simulink model "QD2_Sim_Dual"  (R2025a)
settings: Solver=FixedStepDiscrete  StartTime=0.0  StopTime=400  FixedStep=0.002  RelTol=1e-3
PreLoadFcn:
  | % QD2_Sim_Dual: agrega lib/ y sim/ al path antes de cargar (enlaces a QD2_Mission_Lib)
  | qd2_c = {pwd};
  | qd2_w = which('QD2_Sim_Dual');
  | if ~isempty(qd2_w), qd2_c{end+1} = fileparts(qd2_w); end
  | for qd2_i = 1:numel(qd2_c)
  |     qd2_d = qd2_c{qd2_i};
  |     for qd2_k = 1:4
  |         if exist(fullfile(qd2_d, 'lib', 'QD2_Mission_Lib.slx'), 'file')
  |             addpath(fullfile(qd2_d, 'lib'));
  |             addpath(fullfile(qd2_d, 'sim'));
  |             break;
  |         end
  |         qd2_d = fileparts(qd2_d);
  |     end
  | end
  | clear qd2_c qd2_w qd2_i qd2_d qd2_k
PostLoadFcn:
  | % QD2_Sim_Dual: rutas de lib/ (funciones qd2_* y QD2_Mission_Lib) y sim/
  | qd2_d = fileparts(get_param(bdroot, 'FileName'));
  | for qd2_k = 1:4
  |     if exist(fullfile(qd2_d, 'lib', 'qd2_params.m'), 'file'), break; end
  |     qd2_d = fileparts(qd2_d);
  | end
  | addpath(fullfile(qd2_d, 'lib'));
  | addpath(fullfile(qd2_d, 'sim'));
  | clear qd2_d qd2_k
InitFcn:
  | % QD2_Sim_Dual: rutas de lib/ (funciones qd2_* y QD2_Mission_Lib) y sim/
  | qd2_d = fileparts(get_param(bdroot, 'FileName'));
  | for qd2_k = 1:4
  |     if exist(fullfile(qd2_d, 'lib', 'qd2_params.m'), 'file'), break; end
  |     qd2_d = fileparts(qd2_d);
  | end
  | addpath(fullfile(qd2_d, 'lib'));
  | addpath(fullfile(qd2_d, 'sim'));
  | clear qd2_d qd2_k
  | % Parámetros (config/estacion.json es la única fuente de verdad)
  | QD2P = qd2_params_from_config();
  | QD2_SIM = qd2_sim_parametros();
  | % La versión la fija el bloque constante VERSION de la raíz
  | QD2_VERSION = str2double(get_param([bdroot '/' sprintf('VERSION\n(1 = PID, 2 = MPC)')], 'Value'));
libraries: QD2_Mission_Lib x11, quarc_library x2, simulink x1
settings Model: ExtModeTrigDuration=10000  Creator=ezequ  LastModifiedBy=ezequ
settings SolverCC: AlgebraicLoopSolver=TrustRegion  PositivePriorityOrder=on
settings DataIOCC: SaveFormat=Array  SaveOutput=off  SignalLogging=off  SaveTime=off
settings OptimizationCC: LifeSpan=inf
settings DebuggingCC: AlgebraicLoopMsg=error  UnconnectedInputMsg=warning  UnconnectedOutputMsg=warning  UnconnectedLineMsg=warning  ArithmeticOperatorsInVariantConditions=warning
settings ModelReferenceCC: EnableRefExpFcnMdlSchedulingChecks=on
settings SFSimCC: SimUseLocalCustomCode=off  CustomCodeUndefinedFunction=UseInterfaceOnly
settings RTWCC: SystemTargetFile=quarc_win64.tlc  TemplateMakefile=quarc_default_tmf  RTWUseLocalCustomCode=off  GPUComputeCapability=3.5  Description=QUARC Win64 Target
settings CodeAppCC: StateflowObjectComments=on
settings STFCustomTargetCC: SystemTargetFile=quarc_win64.tlc  TargetPreCompLibLocation=C:\PROGRA~3\QUARC\lib\2016a\win64\release  TargetLangStandard=C99 (ISO)  MultiwordLength=2048.0  DynamicStringBufferSize=256.0  ConcurrentExecutionCompliant=on  Debug=off  StopOnOverrun=off  DownloadToTarget=on
settings GRTTargetCC: ExtMode=on  ExtModeMexFile=quarc_comm  TargetPreCompLibLocation=C:\PROGRA~3\QUARC\lib\2016a\win64\release  ParMdlRefBuildCompliant=off  CompOptLevelCompliant=off  CombineOutputUpdateFcns=off  MatFileLogging=off  CPPClassGenCompliant=off  GRTInterface=on  UseToolchainInfoCompliant=off
settings ConfigComp: CovMetricSettings=dswe

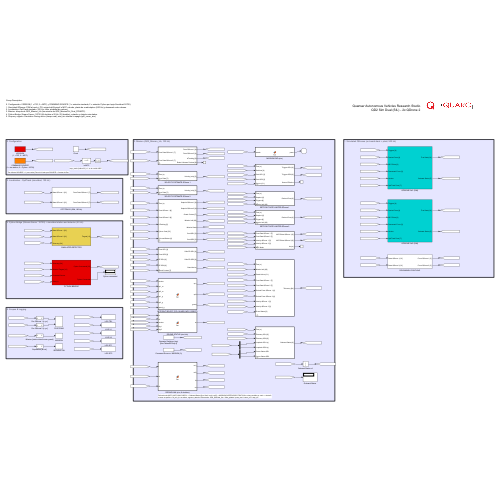
[thumbnail: Simulink's stored preview of the top-level diagram]
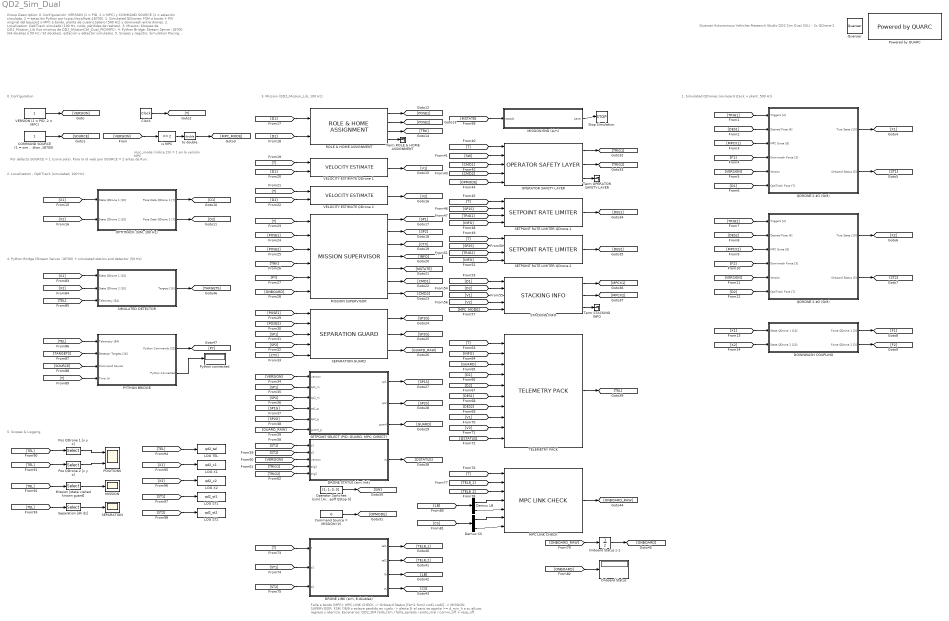
== system QD2_Sim_Dual ==
  note: Group Description:
      |
      | 0. Configuración: VERSION (1 = PID, 2 = MPC) y COMMAND SOURCE (1 = estación simulada, 2 = estación Python por tcpip://localhost:18700).
      | 1. Simulated QDrones: FSM a bordo + PIV original del Equipo2 o MPC a bordo, planta de cuadricóptero (500 Hz) y downwash entre drones.
      | 2. Localization: OptiTrack simulado (100 Hz, ruido, pérdidas de rastreo).
      | 3. Mission: bloques de QD2_Mission_Lib (los mismos de QD2_MissionCtrl_Dual_PID/MPC).
      | 4. Python Bridge: Stream Server :18700 (64 doubles a 50 Hz / 32 doubles), estación y detector simulados.
      | 5. Scopes y registro. Simulation Pacing activo (tiempo real); sim() sin interfaz lo apaga (qd2_correr_sim).
  note: Quanser Autonomous Vehicles Research Studio
      | QD2 Sim Dual (SIL) - 2x QDrone 2
  note: 0. Configuration
  note: mpc_mode (índice 23) = 1 en la versión MPC
  note: Por defecto SOURCE = 1 (corre sola). Para la UI web pon SOURCE = 2 antes de Run.
  note: 1. Simulated QDrones (on-board stack + plant, 500 Hz)
  note: 2. Localization - OptiTrack (simulated, 100 Hz)
  note: 3. Mission (QD2_Mission_Lib, 100 Hz)
  note: Falla a bordo (MPC): MPC LINK CHECK -> Onboard Status [fsm1 fsm2 cod1 cod2] -> MISSION SUPERVISOR. FSM 7/8/9 o enlace perdido en vuelo -> alerta 9:
      | el sano se aparta >= d_min_h a su altura, regresa y aterriza. Escenarios: QD2_SIM.falla_fsm / falla_apilado / proto_mal / comm_off + resp_off.
  note: 4. Python Bridge (Stream Server :18700) + simulated station and detector (50 Hz)
  note: 5. Scopes & Logging
  "COMMAND SOURCE (1 = sim station, 2 = Python :18700)" : Constant
  Clock : DigitalClock  SampleTime=0.01
  Command Source = MISSION (0) : Constant  Value=0  SampleTime=0.01
  DOWNWASH COUPLING : Subsystem
  "DRONE LINK (sim, 8 doubles)" : MATLAB Function  TreatAsAtomicUnit=on
  DRONE STATUS (sim link) : MATLAB Function  TreatAsAtomicUnit=on
  Demux CS : Demux  Outputs=2
  Demux LB : Demux  Outputs=2
  LOG ST1 : ToWorkspace  VariableName=qd2_st1  SampleTime=0.02
  LOG ST2 : ToWorkspace  VariableName=qd2_st2  SampleTime=0.02
  LOG TEL : ToWorkspace  VariableName=qd2_tel  SampleTime=0.02
  LOG X1 : ToWorkspace  VariableName=qd2_x1  SampleTime=0.02
  LOG X2 : ToWorkspace  VariableName=qd2_x2  SampleTime=0.02
  MISSION : Scope
  MISSION END (sim) : MATLAB Function  TreatAsAtomicUnit=on
  MISSION SUPERVISOR : QD2_Mission_Lib/MISSION SUPERVISOR  P=QD2P  version=QD2_VERSION  Ts=0.01
  MPC LINK CHECK : QD2_Mission_Lib/MPC LINK CHECK  P=QD2P  version=QD2_VERSION  Ts=0.01
  Mission [state visited known guard] : Selector  InputPortWidth=64  IndexOptions=Index vector (dialog)  Indices=[2 10 9 11]  OutputSizes=1
  OPERATOR SAFETY LAYER : QD2_Mission_Lib/OPERATOR SAFETY LAYER  Ts=0.01
  "OPTITRACK (SIM, 100 Hz)" : Subsystem
  Onboard Status : Display
  Onboard Status z-1 : UnitDelay  InitialCondition=[0; 0; 0; 0]  SampleTime=0.01  HasFrameUpgradeWarning=on
  Operator Switches (sim) [Arm Takeoff EStop 0] : Constant  Value=[1; 1; 0; 0]  SampleTime=0.01
  POSITIONS : Scope  NumInputPorts=2
  PYTHON BRIDGE : Subsystem
  Pos QDrone 1 [x y z] : Selector  InputPortWidth=64  IndexOptions=Index vector (dialog)  Indices=[17 18 19]  OutputSizes=1
  Pos QDrone 2 [x y z] : Selector  InputPortWidth=64  IndexOptions=Index vector (dialog)  Indices=[35 36 37]  OutputSizes=1
  Powered by QUARC : quarc_library/Logos/Powered by QUARC
  Python connected : Display
  QDRONE 2 #1 (SIM) : Subsystem
  QDRONE 2 #2 (SIM) : Subsystem
  Quanser : quarc_library/Logos/Quanser
  ROLE & HOME ASSIGNMENT : QD2_Mission_Lib/ROLE & HOME ASSIGNMENT  P=QD2P  version=QD2_VERSION  Ts=0.01
  SEPARATION : Scope
  SEPARATION GUARD : QD2_Mission_Lib/SEPARATION GUARD  P=QD2P  Ts=0.01
  SETPOINT RATE LIMITER QDrone 1 : QD2_Mission_Lib/SETPOINT RATE LIMITER  P=QD2P  dron=1  Ts=0.01
  SETPOINT RATE LIMITER QDrone 2 : QD2_Mission_Lib/SETPOINT RATE LIMITER  P=QD2P  dron=2  Ts=0.01
  "SETPOINT SELECT (PID: GUARD, MPC: DIRECT)" : MATLAB Function  TreatAsAtomicUnit=on
  SIMULATED DETECTOR : Subsystem
  STACKING INFO : QD2_Mission_Lib/STACKING INFO  Ts=0.01
  Separation [dh dz] : Selector  InputPortWidth=64  IndexOptions=Index vector (dialog)  Indices=[12 13]  OutputSizes=1
  Stop Simulation : Stop
  TELEMETRY PACK : QD2_Mission_Lib/TELEMETRY PACK  version=QD2_VERSION  Ts=0.01
  Term OPERATOR SAFETY LAYER : Terminator
  Term ROLE & HOME ASSIGNMENT : Terminator
  Term STACKING INFO : Terminator
  VELOCITY ESTIMATE QDrone 1 : QD2_Mission_Lib/VELOCITY ESTIMATE  Ts=0.01
  VELOCITY ESTIMATE QDrone 2 : QD2_Mission_Lib/VELOCITY ESTIMATE  Ts=0.01
  "VERSION (1 = PID, 2 = MPC)" : Constant
  is MPC : simulink/Logic and Bit Operations/Compare To Constant  relop===  const=2  OutDataTypeStr=boolean
  to double : DataTypeConversion  OutDataTypeStr=double  SaturateOnIntegerOverflow=off  RndMeth=Floor
  wires:
  "VERSION (1 = PID, 2 = MPC)"/1 -> [VERSION]
  "COMMAND SOURCE (1 = sim station, 2 = Python :18700)"/1 -> [SOURCE]
  Clock/1 -> [T]
  is MPC/1 -> to double/1
  [VERSION] -> is MPC/1
  to double/1 -> [MPC_MODE]
  [TRIG1] -> QDRONE 2 #1 (SIM)/1(Triggers [4])
  [DES1] -> QDRONE 2 #1 (SIM)/2(Desired Pose [4])
  [MPCX1] -> QDRONE 2 #1 (SIM)/3(MPC Extra [8])
  [F1] -> QDRONE 2 #1 (SIM)/4(Downwash Force [3])
  [VERSION] -> QDRONE 2 #1 (SIM)/5(Version)
  [D1] -> QDRONE 2 #1 (SIM)/6(OptiTrack Pose [7])
  QDRONE 2 #1 (SIM)/1(True State [10]) -> [X1]
  QDRONE 2 #1 (SIM)/2(Onboard Status [5]) -> [ST1]
  [TRIG2] -> QDRONE 2 #2 (SIM)/1(Triggers [4])
  [DES2] -> QDRONE 2 #2 (SIM)/2(Desired Pose [4])
  [MPCX2] -> QDRONE 2 #2 (SIM)/3(MPC Extra [8])
  [F2] -> QDRONE 2 #2 (SIM)/4(Downwash Force [3])
  [VERSION] -> QDRONE 2 #2 (SIM)/5(Version)
  [D2] -> QDRONE 2 #2 (SIM)/6(OptiTrack Pose [7])
  QDRONE 2 #2 (SIM)/1(True State [10]) -> [X2]
  QDRONE 2 #2 (SIM)/2(Onboard Status [5]) -> [ST2]
  [X1] -> DOWNWASH COUPLING/1(State QDrone 1 [10])
  [X2] -> DOWNWASH COUPLING/2(State QDrone 2 [10])
  DOWNWASH COUPLING/1(Force QDrone 1 [3]) -> [F1]
  DOWNWASH COUPLING/2(Force QDrone 2 [3]) -> [F2]
  [X1] -> "OPTITRACK (SIM, 100 Hz)"/1(State QDrone 1 [10])
  [X2] -> "OPTITRACK (SIM, 100 Hz)"/2(State QDrone 2 [10])
  "OPTITRACK (SIM, 100 Hz)"/1(Pose Data QDrone 1 [7]) -> [D1]
  "OPTITRACK (SIM, 100 Hz)"/2(Pose Data QDrone 2 [7]) -> [D2]
  [D1] -> ROLE & HOME ASSIGNMENT/1
  [D2] -> ROLE & HOME ASSIGNMENT/2
  ROLE & HOME ASSIGNMENT/1 -> [POSE1]
  ROLE & HOME ASSIGNMENT/2 -> [POSE2]
  ROLE & HOME ASSIGNMENT/3 -> [TRK]
  ROLE & HOME ASSIGNMENT/4 -> Term ROLE & HOME ASSIGNMENT/1
  [T] -> VELOCITY ESTIMATE QDrone 1/1
  [D1] -> VELOCITY ESTIMATE QDrone 1/2
  VELOCITY ESTIMATE QDrone 1/1 -> [V1]
  [T] -> VELOCITY ESTIMATE QDrone 2/1
  [D2] -> VELOCITY ESTIMATE QDrone 2/2
  VELOCITY ESTIMATE QDrone 2/1 -> [V2]
  [T] -> MISSION SUPERVISOR/1
  [POSE1] -> MISSION SUPERVISOR/2
  [POSE2] -> MISSION SUPERVISOR/3
  [TRK] -> MISSION SUPERVISOR/4
  [PY] -> MISSION SUPERVISOR/5
  [ONBOARD] -> MISSION SUPERVISOR/6
  MISSION SUPERVISOR/1 -> [SP1]
  MISSION SUPERVISOR/2 -> [SP2]
  MISSION SUPERVISOR/3 -> [CTX]
  MISSION SUPERVISOR/4 -> [INFO]
  MISSION SUPERVISOR/5 -> [MSTATE]
  MISSION SUPERVISOR/6 -> [CMD1]
  MISSION SUPERVISOR/7 -> [CMD2]
  [POSE1] -> SEPARATION GUARD/1
  [POSE2] -> SEPARATION GUARD/2
  [SP1] -> SEPARATION GUARD/3
  [SP2] -> SEPARATION GUARD/4
  [CTX] -> SEPARATION GUARD/5
  SEPARATION GUARD/1 -> [SP1G]
  SEPARATION GUARD/2 -> [SP2G]
  SEPARATION GUARD/3 -> [GUARD_RAW]
  [VERSION] -> "SETPOINT SELECT (PID: GUARD, MPC: DIRECT)"/1(version)
  [SP1] -> "SETPOINT SELECT (PID: GUARD, MPC: DIRECT)"/2(sp1_m)
  [SP2] -> "SETPOINT SELECT (PID: GUARD, MPC: DIRECT)"/3(sp2_m)
  [SP1G] -> "SETPOINT SELECT (PID: GUARD, MPC: DIRECT)"/4(sp1_g)
  [SP2G] -> "SETPOINT SELECT (PID: GUARD, MPC: DIRECT)"/5(sp2_g)
  [GUARD_RAW] -> "SETPOINT SELECT (PID: GUARD, MPC: DIRECT)"/6(guard_g)
  "SETPOINT SELECT (PID: GUARD, MPC: DIRECT)"/1(sp1) -> [SP1S]
  "SETPOINT SELECT (PID: GUARD, MPC: DIRECT)"/2(sp2) -> [SP2S]
  "SETPOINT SELECT (PID: GUARD, MPC: DIRECT)"/3(guard) -> [GUARD]
  Operator Switches (sim) [Arm Takeoff EStop 0]/1 -> [SW]
  Command Source = MISSION (0)/1 -> [OPMODE]
  [T] -> OPERATOR SAFETY LAYER/1
  [SW] -> OPERATOR SAFETY LAYER/2
  [CMD1] -> OPERATOR SAFETY LAYER/3
  [CMD2] -> OPERATOR SAFETY LAYER/4
  [OPMODE] -> OPERATOR SAFETY LAYER/5
  OPERATOR SAFETY LAYER/1 -> [TRIG1]
  OPERATOR SAFETY LAYER/2 -> [TRIG2]
  OPERATOR SAFETY LAYER/3 -> Term OPERATOR SAFETY LAYER/1
  [T] -> SETPOINT RATE LIMITER QDrone 1/1
  [SP1S] -> SETPOINT RATE LIMITER QDrone 1/2
  [TRIG1] -> SETPOINT RATE LIMITER QDrone 1/3
  [INFO] -> SETPOINT RATE LIMITER QDrone 1/4
  SETPOINT RATE LIMITER QDrone 1/1 -> [DES1]
  [T] -> SETPOINT RATE LIMITER QDrone 2/1
  [SP2S] -> SETPOINT RATE LIMITER QDrone 2/2
  [TRIG2] -> SETPOINT RATE LIMITER QDrone 2/3
  [INFO] -> SETPOINT RATE LIMITER QDrone 2/4
  SETPOINT RATE LIMITER QDrone 2/1 -> [DES2]
  [D1] -> STACKING INFO/1
  [D2] -> STACKING INFO/2
  [V1] -> STACKING INFO/3
  [V2] -> STACKING INFO/4
  [MPC_MODE] -> STACKING INFO/5
  STACKING INFO/1 -> [MPCX1]
  STACKING INFO/2 -> [MPCX2]
  STACKING INFO/3 -> Term STACKING INFO/1
  [ST1] -> DRONE STATUS (sim link)/1(s1)
  [ST2] -> DRONE STATUS (sim link)/2(s2)
  [VERSION] -> DRONE STATUS (sim link)/3(version)
  [TRIG1] -> DRONE STATUS (sim link)/4(trig1)
  [TRIG2] -> DRONE STATUS (sim link)/5(trig2)
  DRONE STATUS (sim link)/1(st) -> [DSTATUS]
  [T] -> TELEMETRY PACK/1
  [INFO] -> TELEMETRY PACK/2
  [GUARD] -> TELEMETRY PACK/3
  [D1] -> TELEMETRY PACK/4
  [D2] -> TELEMETRY PACK/5
  [DES1] -> TELEMETRY PACK/6
  [DES2] -> TELEMETRY PACK/7
  [V1] -> TELEMETRY PACK/8
  [V2] -> TELEMETRY PACK/9
  [DSTATUS] -> TELEMETRY PACK/10
  TELEMETRY PACK/1 -> [TEL]
  [T] -> "DRONE LINK (sim, 8 doubles)"/1(t)
  [ST1] -> "DRONE LINK (sim, 8 doubles)"/2(s1)
  [ST2] -> "DRONE LINK (sim, 8 doubles)"/3(s2)
  "DRONE LINK (sim, 8 doubles)"/1(tel1) -> [TEL8_1]
  "DRONE LINK (sim, 8 doubles)"/2(tel2) -> [TEL8_2]
  "DRONE LINK (sim, 8 doubles)"/3(lb) -> [LB]
  "DRONE LINK (sim, 8 doubles)"/4(cs) -> [CS]
  [T] -> MPC LINK CHECK/1
  [TEL8_1] -> MPC LINK CHECK/2
  [TEL8_2] -> MPC LINK CHECK/3
  MPC LINK CHECK/1 -> [ONBOARD_RAW]
  [ONBOARD_RAW] -> Onboard Status z-1/1
  Onboard Status z-1/1 -> [ONBOARD]
  [LB] -> Demux LB/1
  Demux LB/1 -> MPC LINK CHECK/4
  Demux LB/2 -> MPC LINK CHECK/5
  [CS] -> Demux CS/1
  Demux CS/1 -> MPC LINK CHECK/6
  Demux CS/2 -> MPC LINK CHECK/7
  [ONBOARD] -> Onboard Status/1
  [X1] -> SIMULATED DETECTOR/1(State QDrone 1 [10])
  [X2] -> SIMULATED DETECTOR/2(State QDrone 2 [10])
  [TEL] -> SIMULATED DETECTOR/3(Telemetry [64])
  SIMULATED DETECTOR/1(Targets [16]) -> [TARGETS]
  [TEL] -> PYTHON BRIDGE/1(Telemetry [64])
  [TARGETS] -> PYTHON BRIDGE/2(Detector Targets [16])
  [SOURCE] -> PYTHON BRIDGE/3(Command Source)
  [T] -> PYTHON BRIDGE/4(Time (s))
  PYTHON BRIDGE/1(Python Commands [32]) -> [PY]
  PYTHON BRIDGE/2(Python Connected) -> Python connected/1
  [TEL] -> Pos QDrone 1 [x y z]/1
  [TEL] -> Pos QDrone 2 [x y z]/1
  [TEL] -> Mission [state visited known guard]/1
  [TEL] -> Separation [dh dz]/1
  Pos QDrone 1 [x y z]/1 -> POSITIONS/1
  Pos QDrone 2 [x y z]/1 -> POSITIONS/2
  Mission [state visited known guard]/1 -> MISSION/1
  Separation [dh dz]/1 -> SEPARATION/1
  [TEL] -> LOG TEL/1
  [X1] -> LOG X1/1
  [X2] -> LOG X2/1
  [ST1] -> LOG ST1/1
  [ST2] -> LOG ST2/1
  [MSTATE] -> MISSION END (sim)/1(estado)
  MISSION END (sim)/1(parar) -> Stop Simulation/1

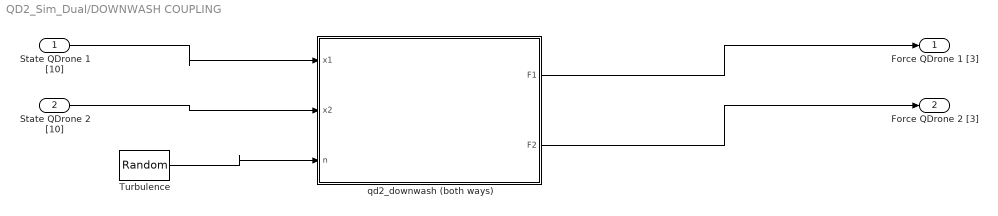
== system QD2_Sim_Dual/DOWNWASH COUPLING ==
  State QDrone 1 [10] : Inport
  State QDrone 2 [10] : Inport  Port=2
  Turbulence : RandomNumber  Mean=zeros(6,1)  Variance=ones(6,1)  Seed=QD2_SIM.semilla + [11 12 13 14 15 16]'  SampleTime=0.002
  qd2_downwash (both ways) : MATLAB Function  TreatAsAtomicUnit=on
  Force QDrone 1 [3] : Outport
  Force QDrone 2 [3] : Outport  Port=2
  wires:
  State QDrone 1 [10]/1 -> qd2_downwash (both ways)/1(x1)
  State QDrone 2 [10]/1 -> qd2_downwash (both ways)/2(x2)
  Turbulence/1 -> qd2_downwash (both ways)/3(n)
  qd2_downwash (both ways)/1(F1) -> Force QDrone 1 [3]/1
  qd2_downwash (both ways)/2(F2) -> Force QDrone 2 [3]/1

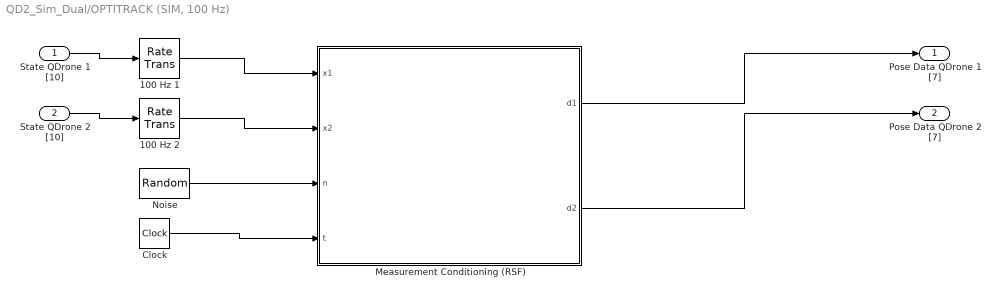
== system QD2_Sim_Dual/OPTITRACK (SIM, 100 Hz) ==
  State QDrone 1 [10] : Inport
  State QDrone 2 [10] : Inport  Port=2
  100 Hz 1 : RateTransition  OutPortSampleTime=0.01
  100 Hz 2 : RateTransition  OutPortSampleTime=0.01
  Clock : DigitalClock  SampleTime=0.01
  Measurement Conditioning (RSF) : MATLAB Function  TreatAsAtomicUnit=on
  Noise : RandomNumber  Mean=zeros(8,1)  Variance=ones(8,1)  Seed=QD2_SIM.semilla + (21:28)'  SampleTime=0.01
  Pose Data QDrone 1 [7] : Outport
  Pose Data QDrone 2 [7] : Outport  Port=2
  wires:
  State QDrone 1 [10]/1 -> 100 Hz 1/1
  State QDrone 2 [10]/1 -> 100 Hz 2/1
  100 Hz 1/1 -> Measurement Conditioning (RSF)/1(x1)
  100 Hz 2/1 -> Measurement Conditioning (RSF)/2(x2)
  Noise/1 -> Measurement Conditioning (RSF)/3(n)
  Clock/1 -> Measurement Conditioning (RSF)/4(t)
  Measurement Conditioning (RSF)/1(d1) -> Pose Data QDrone 1 [7]/1
  Measurement Conditioning (RSF)/2(d2) -> Pose Data QDrone 2 [7]/1

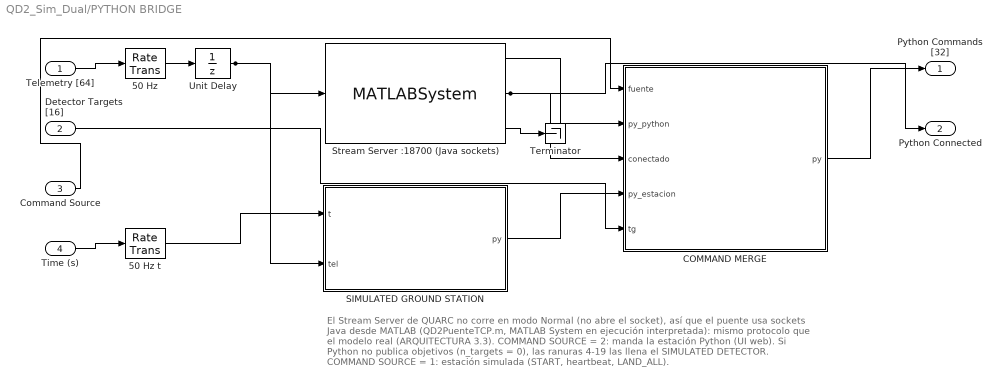
== system QD2_Sim_Dual/PYTHON BRIDGE ==
  note: El Stream Server de QUARC no corre en modo Normal (no abre el socket), así que el puente usa sockets Java desde MATLAB
      | (QD2PuenteTCP.m, MATLAB System en ejecución interpretada): mismo protocolo que el modelo real (ARQUITECTURA 3.3).
      | COMMAND SOURCE = 2: manda la estación Python (UI web). Si Python no publica objetivos (n_targets = 0), las
      | ranuras 4-19 las llena el SIMULATED DETECTOR. COMMAND SOURCE = 1: estación simulada (START, heartbeat, LAND_ALL).
  Telemetry [64] : Inport
  Detector Targets [16] : Inport  Port=2
  Command Source : Inport  Port=3
  Time (s) : Inport  Port=4
  50 Hz : RateTransition  OutPortSampleTime=0.02
  50 Hz t : RateTransition  OutPortSampleTime=0.02
  COMMAND MERGE : MATLAB Function  TreatAsAtomicUnit=on
  SIMULATED GROUND STATION : MATLAB Function  TreatAsAtomicUnit=on
  Stream Server :18700 (Java sockets) : MATLABSystem  System=QD2PuenteTCP  Puerto=QD2_SIM.puerto  Direccion=127.0.0.1  Activo=1  TDesconectar=5  Ts=0.02
      mask Type: QD2PuenteTCP
  Terminator : Terminator
  Unit Delay : UnitDelay  InitialCondition=zeros(64,1)  SampleTime=0.02  HasFrameUpgradeWarning=on
  Python Commands [32] : Outport
  Python Connected : Outport  Port=2
  wires:
  Telemetry [64]/1 -> 50 Hz/1
  50 Hz/1 -> Unit Delay/1
  Unit Delay/1 -> Stream Server :18700 (Java sockets)/1, SIMULATED GROUND STATION/2(tel)
  Time (s)/1 -> 50 Hz t/1
  50 Hz t/1 -> SIMULATED GROUND STATION/1(t)
  Command Source/1 -> COMMAND MERGE/1(fuente)
  Stream Server :18700 (Java sockets)/1 -> COMMAND MERGE/2(py_python)
  Stream Server :18700 (Java sockets)/2 -> COMMAND MERGE/3(conectado), Python Connected/1
  SIMULATED GROUND STATION/1(py) -> COMMAND MERGE/4(py_estacion)
  Detector Targets [16]/1 -> COMMAND MERGE/5(tg)
  COMMAND MERGE/1(py) -> Python Commands [32]/1
  Stream Server :18700 (Java sockets)/3 -> Terminator/1

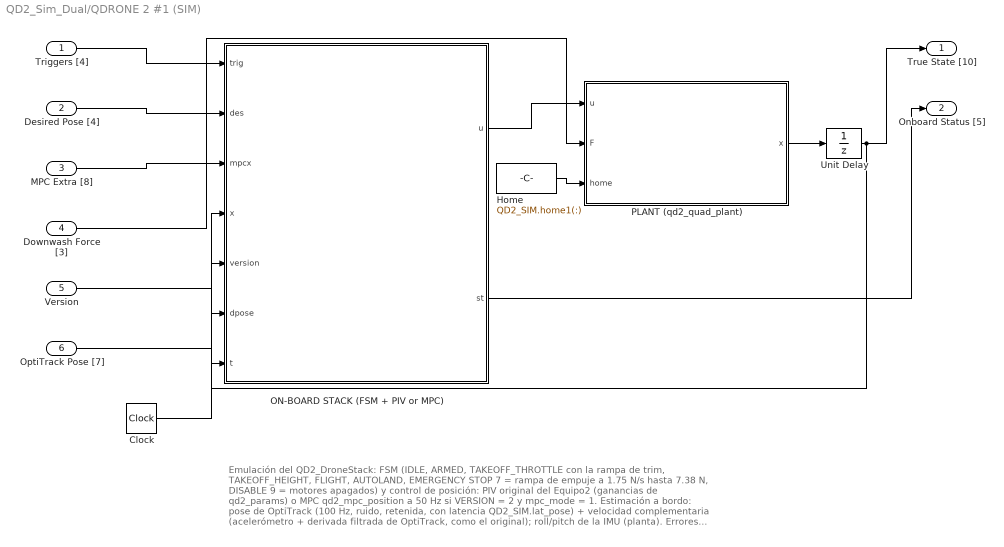
== system QD2_Sim_Dual/QDRONE 2 #1 (SIM) ==
  note: Emulación del QD2_DroneStack: FSM (IDLE, ARMED, TAKEOFF_THROTTLE con la rampa de trim, TAKEOFF_HEIGHT, FLIGHT, AUTOLAND,
      | EMERGENCY STOP 7 = rampa de empuje a 1.75 N/s hasta 7.38 N, DISABLE 9 = motores apagados) y control de posición: PIV original del
      | Equipo2 (ganancias de qd2_params) o MPC qd2_mpc_position a 50 Hz si VERSION = 2 y mpc_mode = 1.
      | Estimación a bordo: pose de OptiTrack (100 Hz, ruido, retenida, con latencia QD2_SIM.lat_pose) + velocidad complementaria
      | (acelerómetro + derivada filtrada de OptiTrack, como el original); roll/pitch de la IMU (planta). Errores como el original:
      | isTracking = 0 durante 0.2 s -> 7; enlace caído (QD2_SIM.comm_off) 0.5 s -> 7 y 1 s armado -> 9 (FLIGHT SAFETY corta motores).
      | Fallas a bordo programadas: QD2_SIM.falla_fsm [dron t] o QD2_SIM.falla_apilado (1 = el de arriba, 2 = el de abajo) -> 7.
      | Onboard Status = [FSM, batería (V), estado MPC (0 ok, 3 inactivo, 4 PIV), empuje (N), comm issue].
      | True State = [x y z vx vy vz roll pitch yaw T]. El STABILIZER se aproxima con la actitud de 1er orden de la planta.
  Triggers [4] : Inport
  Desired Pose [4] : Inport  Port=2
  MPC Extra [8] : Inport  Port=3
  Downwash Force [3] : Inport  Port=4
  Version : Inport  Port=5
  OptiTrack Pose [7] : Inport  Port=6
  Clock : DigitalClock  SampleTime=0.002
  Home : Constant  Value=QD2_SIM.home1(:)
  ON-BOARD STACK (FSM + PIV or MPC) : MATLAB Function  TreatAsAtomicUnit=on
  PLANT (qd2_quad_plant) : MATLAB Function  TreatAsAtomicUnit=on
  Unit Delay : UnitDelay  InitialCondition=[QD2_SIM.home1(:); zeros(8,1)]  SampleTime=0.002  HasFrameUpgradeWarning=on
  True State [10] : Outport
  Onboard Status [5] : Outport  Port=2
  wires:
  Triggers [4]/1 -> ON-BOARD STACK (FSM + PIV or MPC)/1(trig)
  Desired Pose [4]/1 -> ON-BOARD STACK (FSM + PIV or MPC)/2(des)
  MPC Extra [8]/1 -> ON-BOARD STACK (FSM + PIV or MPC)/3(mpcx)
  Unit Delay/1 -> ON-BOARD STACK (FSM + PIV or MPC)/4(x), True State [10]/1
  Version/1 -> ON-BOARD STACK (FSM + PIV or MPC)/5(version)
  OptiTrack Pose [7]/1 -> ON-BOARD STACK (FSM + PIV or MPC)/6(dpose)
  Clock/1 -> ON-BOARD STACK (FSM + PIV or MPC)/7(t)
  ON-BOARD STACK (FSM + PIV or MPC)/1(u) -> PLANT (qd2_quad_plant)/1(u)
  Downwash Force [3]/1 -> PLANT (qd2_quad_plant)/2(F)
  Home/1 -> PLANT (qd2_quad_plant)/3(home)
  PLANT (qd2_quad_plant)/1(x) -> Unit Delay/1
  ON-BOARD STACK (FSM + PIV or MPC)/2(st) -> Onboard Status [5]/1

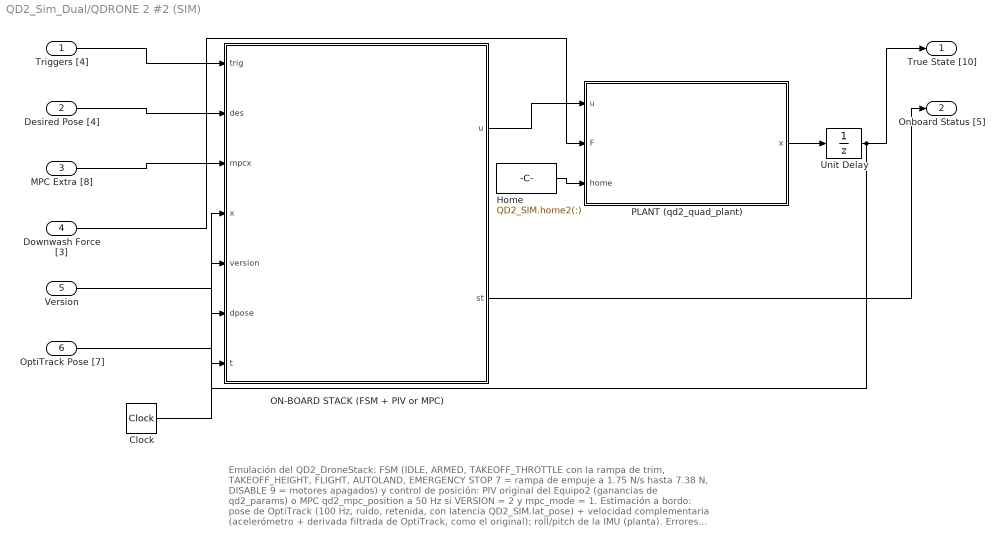
== system QD2_Sim_Dual/QDRONE 2 #2 (SIM) ==
  note: Emulación del QD2_DroneStack: FSM (IDLE, ARMED, TAKEOFF_THROTTLE con la rampa de trim, TAKEOFF_HEIGHT, FLIGHT, AUTOLAND,
      | EMERGENCY STOP 7 = rampa de empuje a 1.75 N/s hasta 7.38 N, DISABLE 9 = motores apagados) y control de posición: PIV original del
      | Equipo2 (ganancias de qd2_params) o MPC qd2_mpc_position a 50 Hz si VERSION = 2 y mpc_mode = 1.
      | Estimación a bordo: pose de OptiTrack (100 Hz, ruido, retenida, con latencia QD2_SIM.lat_pose) + velocidad complementaria
      | (acelerómetro + derivada filtrada de OptiTrack, como el original); roll/pitch de la IMU (planta). Errores como el original:
      | isTracking = 0 durante 0.2 s -> 7; enlace caído (QD2_SIM.comm_off) 0.5 s -> 7 y 1 s armado -> 9 (FLIGHT SAFETY corta motores).
      | Fallas a bordo programadas: QD2_SIM.falla_fsm [dron t] o QD2_SIM.falla_apilado (1 = el de arriba, 2 = el de abajo) -> 7.
      | Onboard Status = [FSM, batería (V), estado MPC (0 ok, 3 inactivo, 4 PIV), empuje (N), comm issue].
      | True State = [x y z vx vy vz roll pitch yaw T]. El STABILIZER se aproxima con la actitud de 1er orden de la planta.
  Triggers [4] : Inport
  Desired Pose [4] : Inport  Port=2
  MPC Extra [8] : Inport  Port=3
  Downwash Force [3] : Inport  Port=4
  Version : Inport  Port=5
  OptiTrack Pose [7] : Inport  Port=6
  Clock : DigitalClock  SampleTime=0.002
  Home : Constant  Value=QD2_SIM.home2(:)
  ON-BOARD STACK (FSM + PIV or MPC) : MATLAB Function  TreatAsAtomicUnit=on
  PLANT (qd2_quad_plant) : MATLAB Function  TreatAsAtomicUnit=on
  Unit Delay : UnitDelay  InitialCondition=[QD2_SIM.home2(:); zeros(8,1)]  SampleTime=0.002  HasFrameUpgradeWarning=on
  True State [10] : Outport
  Onboard Status [5] : Outport  Port=2
  wires:
  Triggers [4]/1 -> ON-BOARD STACK (FSM + PIV or MPC)/1(trig)
  Desired Pose [4]/1 -> ON-BOARD STACK (FSM + PIV or MPC)/2(des)
  MPC Extra [8]/1 -> ON-BOARD STACK (FSM + PIV or MPC)/3(mpcx)
  Unit Delay/1 -> ON-BOARD STACK (FSM + PIV or MPC)/4(x), True State [10]/1
  Version/1 -> ON-BOARD STACK (FSM + PIV or MPC)/5(version)
  OptiTrack Pose [7]/1 -> ON-BOARD STACK (FSM + PIV or MPC)/6(dpose)
  Clock/1 -> ON-BOARD STACK (FSM + PIV or MPC)/7(t)
  ON-BOARD STACK (FSM + PIV or MPC)/1(u) -> PLANT (qd2_quad_plant)/1(u)
  Downwash Force [3]/1 -> PLANT (qd2_quad_plant)/2(F)
  Home/1 -> PLANT (qd2_quad_plant)/3(home)
  PLANT (qd2_quad_plant)/1(x) -> Unit Delay/1
  ON-BOARD STACK (FSM + PIV or MPC)/2(st) -> Onboard Status [5]/1

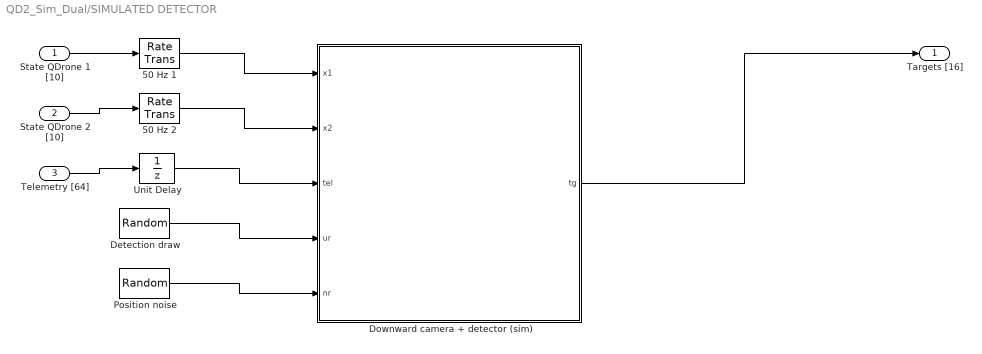
== system QD2_Sim_Dual/SIMULATED DETECTOR ==
  State QDrone 1 [10] : Inport
  State QDrone 2 [10] : Inport  Port=2
  Telemetry [64] : Inport  Port=3
  50 Hz 1 : RateTransition  OutPortSampleTime=0.02
  50 Hz 2 : RateTransition  OutPortSampleTime=0.02
  Detection draw : UniformRandomNumber  Minimum=zeros(16,1)  Maximum=ones(16,1)  Seed=QD2_SIM.semilla + (31:46)'  SampleTime=0.02
  Downward camera + detector (sim) : MATLAB Function  TreatAsAtomicUnit=on
  Position noise : RandomNumber  Mean=zeros(2,1)  Variance=ones(2,1)  Seed=QD2_SIM.semilla + [51; 52]  SampleTime=0.02
  Unit Delay : UnitDelay  InitialCondition=zeros(64,1)  SampleTime=0.02  HasFrameUpgradeWarning=on
  Targets [16] : Outport
  wires:
  State QDrone 1 [10]/1 -> 50 Hz 1/1
  State QDrone 2 [10]/1 -> 50 Hz 2/1
  Telemetry [64]/1 -> Unit Delay/1
  50 Hz 1/1 -> Downward camera + detector (sim)/1(x1)
  50 Hz 2/1 -> Downward camera + detector (sim)/2(x2)
  Unit Delay/1 -> Downward camera + detector (sim)/3(tel)
  Detection draw/1 -> Downward camera + detector (sim)/4(ur)
  Position noise/1 -> Downward camera + detector (sim)/5(nr)
  Downward camera + detector (sim)/1(tg) -> Targets [16]/1

== matlab function QD2_Sim_Dual/DRONE STATUS (sim link) ==
  data: s1 input; st output size=[8 1]; s2 input; version input; trig1 input; trig2 input
function st = fcn(s1, s2, version, trig1, trig2)
%#codegen
% Drone Status [8] para el TELEMETRY PACK: [fsm1 fsm2 bat1 bat2 comm_issue1
% comm_issue2 loopback1 loopback2]. comm_issue viene de la emulación a bordo
% (pérdidas programadas QD2_SIM.comm_off); loopback = 0 (sin latencia de red).
% fsm (o+2 de la telemetría, ARQUITECTURA §3.3) según la versión, como los
% modelos de tierra: PID = Flight State de TIERRA (Flight Plan del Equipo2:
% 0 Idle, 1 Armed, 2 Takeoff, 3 Land, 9 MS Stop) con los disparos efectivos
% trig = [arm takeoff estop 0] y comm_issue; MPC = FSM a bordo (1..9).
persistent fp
if isempty(fp)
    fp = [0; 0];
end
fp(1) = flight_plan(fp(1), trig1, s1(5));
fp(2) = flight_plan(fp(2), trig2, s2(5));
if version < 1.5
    f1 = fp(1); f2 = fp(2);
else
    f1 = s1(1); f2 = s2(1);
end
st = [f1; f2; s1(2); s2(2); s1(5); s2(5); 0; 0];
end

function e = flight_plan(e, trig, com)
% Copia de Flight_Plan (QD2_MissionCtrl_NoJoystick_2021a/Subsystem), joystick_issue = 0.
arm = trig(1) > 0.5; tk = trig(2) > 0.5; es = trig(3) > 0.5; ci = com > 0.5;
if e == 0
    if arm && ~es
        e = 1;
    elseif es || tk || ci
        e = 9;
    end
elseif e == 1
    if ~es
        if ~arm
            e = 0;
        elseif tk
            e = 2;
        end
    elseif ci || es
        e = 9;
    end
elseif e == 2
    if ~es
        if ~tk
            e = 3;
        elseif ~arm || ci
            e = 9;
        end
    end
elseif e == 3
    if ~arm || ci
        e = 9;
    end
end
end

== matlab function QD2_Sim_Dual/DRONE LINK (sim, 8 doubles) ==
  data: t input; tel1 output size=[8 1]; s1 input; s2 input; tel2 output size=[8 1]; lb output size=[2 1]; cs output size=[2 1]; QD2_SIM parameter
function [tel1, tel2, lb, cs] = fcn(t, s1, s2, QD2_SIM)
%#codegen
% DRONE LINK (sim): respuesta de 8 doubles de cada dron como la manda
% QD2_DroneStack_MPC (ARQUITECTURA §3.2): [eco ts, FSM, batería, estado MPC, T,
% roll, pitch, 2 = etiqueta protocolo MPC v1]. s1/s2 = Onboard Status [FSM bat est T comm].
% QD2_SIM.proto_mal [dron t1 t2]: ese dron responde sin la etiqueta (0) en [t1, t2).
% QD2_SIM.resp_off [dron t1 t2]: la respuesta dron->PC no llega en [t1, t2): el Stream
% Server ("most recent") retiene la última y el loopback crece (lb = t - eco retenido).
% lb = loopback (0: el enlace simulado no tiene latencia); cs = Communication Status
% (1 si el dron perdió el enlace PC->dron, QD2_SIM.comm_off).
persistent u1 u2
if isempty(u1)
    u1 = [0; NaN(7, 1)];
    u2 = [0; NaN(7, 1)];
end
tg = [2 2];
pm = QD2_SIM.proto_mal;
for k = 1:size(pm, 1)
    if pm(k,1) >= 1 && pm(k,1) <= 2 && t >= pm(k,2) && t < pm(k,3)
        tg(pm(k,1)) = 0;
    end
end
perd = [false false];
ro = QD2_SIM.resp_off;
for k = 1:size(ro, 1)
    if ro(k,1) >= 1 && ro(k,1) <= 2 && t >= ro(k,2) && t < ro(k,3)
        perd(ro(k,1)) = true;
    end
end
lb = [0; 0];
if ~perd(1)
    u1 = [t; s1(1); s1(2); s1(3); s1(4); 0; 0; tg(1)];
else
    lb(1) = t - u1(1);
end
if ~perd(2)
    u2 = [t; s2(1); s2(2); s2(3); s2(4); 0; 0; tg(2)];
else
    lb(2) = t - u2(1);
end
tel1 = u1;
tel2 = u2;
cs = [s1(5); s2(5)];

== matlab function QD2_Sim_Dual/SIMULATED DETECTOR/Downward camera + detector (sim) ==
  data: x1 input; tg output size=[16 1]; x2 input; tel input; ur input; nr input; QD2_SIM parameter
function tg = fcn(x1, x2, tel, ur, nr, QD2_SIM)
%#codegen
% DETECTOR SIMULADO: cámara cenital del EXPLORADOR (RealSense mirando abajo).
% Huella = rectángulo de semiancho z*tan(vfov/2) (eje x del dron) por
% z*tan(hfov/2) (eje y), centrado en la cámara (offset del soporte).
% Cada objetivo dentro de la huella cuenta una observación por frame
% (~12.5 fps) con probabilidad det_p; con det_frames observaciones se
% publica como lo haría la estación Python: [id clase x y confianza].
% Salida tg = [n_targets; 3 ranuras x 5] (índices 4-19 del paquete de 32),
% rotando las ranuras entre todos los publicados.
persistent obs pub npub k rot
if isempty(obs)
    obs = zeros(16, 1);
    pub = zeros(16, 5);
    npub = 0;
    k = 0;
    rot = 0;
end
k = k + 1;
O = QD2_SIM.objetivos_tabla;
eid = tel(4);
estado = tel(2);
if mod(k, 4) == 0 && (eid == 1 || eid == 2) && estado >= 4 && estado <= 6
    if eid == 1
        xe = x1;
    else
        xe = x2;
    end
    z = xe(3);
    if z >= QD2_SIM.det_z_min
        c = cos(xe(9)); s = sin(xe(9));
        cx = xe(1) + c*QD2_SIM.det_offset(1) - s*QD2_SIM.det_offset(2);
        cy = xe(2) + s*QD2_SIM.det_offset(1) + c*QD2_SIM.det_offset(2);
        hx = z*tan(QD2_SIM.det_vfov*pi/360);
        hy = z*tan(QD2_SIM.det_hfov*pi/360);
        for j = 1:16
            if isfinite(O(j,1)) && obs(j) < QD2_SIM.det_frames
                dx = O(j,1) - cx; dy = O(j,2) - cy;
                bx = c*dx + s*dy; by = -s*dx + c*dy;
                if abs(bx) <= hx && abs(by) <= hy && ur(j) < QD2_SIM.det_p
                    obs(j) = obs(j) + 1;
                    if obs(j) >= QD2_SIM.det_frames && npub < 16
                        npub = npub + 1;
                        pub(npub, :) = [npub, O(j,3), O(j,1) + QD2_SIM.det_ruido*nr(1), ...
                                        O(j,2) + QD2_SIM.det_ruido*nr(2), 0.85];
                    end
                end
            end
        end
    end
end
tg = zeros(16, 1);
tg(1) = npub;
if npub > 0
    rot = rot + 1;
    for r = 1:3
        q = mod(rot*3 + r - 1, npub) + 1;
        tg(2 + 5*(r-1) : 6 + 5*(r-1)) = pub(q, :)';
    end
end

== matlab function QD2_Sim_Dual/PYTHON BRIDGE/SIMULATED GROUND STATION ==
  data: t input; py output size=[32 1]; tel input; QD2P parameter; QD2_SIM parameter
function py = fcn(t, tel, QD2P, QD2_SIM)
%#codegen
% ESTACIÓN SIMULADA (para correr sin la UI): heartbeat a 50 Hz, START en
% QD2_SIM.t_start y LAND_ALL cuando los dos drones llevan t_land_espera s en
% su home durante RETURN_HOME (si auto_land = false).
persistent hb seq cmd t_casa start_ok land_ok
if isempty(hb)
    hb = 0; seq = 0; cmd = 0; t_casa = -1; start_ok = 0; land_ok = 0;
end
hb = hb + 1;
estado = tel(2);
if start_ok < 0.5 && t >= QD2_SIM.t_start && estado == 2
    seq = seq + 1; cmd = 1; start_ok = 1;
end
en_casa = false;
if estado == 6
    d1 = hypot(tel(17) - tel(29), tel(18) - tel(30));
    d2 = hypot(tel(35) - tel(47), tel(36) - tel(48));
    en_casa = d1 < 0.15 && d2 < 0.15;
end
if en_casa
    if t_casa < 0, t_casa = t; end
else
    t_casa = -1;
end
if land_ok < 0.5 && QD2P.auto_land < 0.5 && t_casa >= 0 && t - t_casa >= QD2_SIM.t_land_espera
    seq = seq + 1; cmd = 3; land_ok = 1;
end
py = zeros(32, 1);
py(1) = hb;
py(2) = cmd;
py(3) = seq;

== matlab function QD2_Sim_Dual/PYTHON BRIDGE/COMMAND MERGE ==
  data: fuente input; py output size=[32 1]; py_python input; conectado input; py_estacion input; tg input
function py = fcn(fuente, py_python, conectado, py_estacion, tg)
%#codegen
% COMMAND MERGE: elige la fuente de comandos y completa los objetivos.
if fuente > 1.5
    % sin cliente queda el último paquete: el heartbeat deja de crecer
    % (-> PAUSED en MISSION), igual que con el puente real
    py = py_python + 0*conectado;
else
    py = py_estacion;
end
% Si la fuente no publica objetivos, los pone el detector simulado.
if py(4) < 0.5
    py(4) = tg(1);
    for i = 1:15
        py(4 + i) = tg(1 + i);
    end
end

== matlab function QD2_Sim_Dual/QDRONE 2 #1 (SIM)/PLANT (qd2_quad_plant) ==
  data: u input; x output size=[10 1]; F input; home input; QD2P parameter
function x = fcn(u, F, home, QD2P)
%#codegen
% PLANTA: qd2_quad_plant (traslación 3D, actitud y empuje de 1er orden, suelo).
persistent xs
if isempty(xs)
    xs = zeros(10, 1);
    xs(1) = home(1);
    xs(2) = home(2);
end
xs = qd2_quad_plant(xs, u, F, 0.002, QD2P.planta);
x = xs;

== matlab function QD2_Sim_Dual/MISSION END (sim) ==
  data: estado input; parar output size=1; QD2_SIM parameter
function parar = fcn(estado, QD2_SIM)
%#codegen
% Detiene la simulación 3 s después de DONE (si QD2_SIM.parar_en_done = 1).
persistent n
if isempty(n), n = 0; end
if estado == 8
    n = n + 1;
else
    n = 0;
end
parar = double(QD2_SIM.parar_en_done > 0.5 && n >= 300);

== matlab function QD2_Sim_Dual/QDRONE 2 #1 (SIM)/ON-BOARD STACK (FSM + PIV or MPC) ==
  data: trig input; u output size=[4 1]; des input; mpcx input; x input; version input; dpose input; t input; st output size=[5 1]; QD2P parameter; QD2_SIM parameter
function [u, st] = fcn(trig, des, mpcx, x, version, dpose, t, QD2P, QD2_SIM)
%#codegen
% STACK A BORDO SIMULADO del QDrone 2 #1 (500 Hz): FSM + PIV original o MPC
% (qd2_onboard_step), con la estimación y los errores del stack real.
% trig = [arm takeoff estop 0], des = pose deseada [x y z yaw],
% mpcx = [otro dron x y z vx vy vz, mpc_mode, 0] (índices 17-24 del paquete MPC),
% x = estado verdadero de la planta (solo para la IMU: roll, pitch, aceleración),
% dpose = OptiTrack [x y z roll pitch yaw isTracking] (100 Hz, NaN sin rastreo).
ID = 1;
NB = 64;
persistent ob bat buf kb pos vf1 vf2 vest vprev pprev t_trk t_com paq T7 u_prev fh t_ap
dt = 0.002;
if isempty(ob)
    ob = qd2_onboard_init(QD2P);
    bat = 16.4;
    buf = zeros(7, NB);
    for j = 1:NB
        buf(:, j) = [x(1); x(2); x(3); x(7); x(8); x(9); 1];
    end
    kb = 1;
    pos = [x(1); x(2); x(3); x(9)];
    pprev = pos(1:3);
    vf1 = zeros(3, 1); vf2 = zeros(3, 1); vest = zeros(3, 1);
    vprev = [x(4); x(5); x(6)];
    t_trk = 0; t_com = 0; T7 = 0;
    paq = [trig(:); des(:); mpcx(:); dpose(:)];
    u_prev = zeros(4, 1);
    fh = false; t_ap = 0;
end
% ---- enlace PC -> dron: pérdidas programadas QD2_SIM.comm_off [dron t1 t2] ----
sin_enlace = false;
co = QD2_SIM.comm_off;
for k = 1:size(co, 1)
    if co(k,1) == ID && t >= co(k,2) && t < co(k,3)
        sin_enlace = true;
    end
end
if ~sin_enlace
    paq = [trig(:); des(:); mpcx(:); dpose(:)];   % "most recent": sin enlace queda el último
    t_com = 0;
else
    t_com = t_com + dt;
end
tr = paq(1:4); ds = paq(5:8); mx = paq(9:16); dp = paq(17:23);
% ---- estimación a bordo ------------------------------------------------
% pose OptiTrack con latencia (buffer circular a 500 Hz)
buf(:, kb) = dp;
nl = min(max(round(QD2_SIM.lat_pose/dt), 0), NB - 1);
j = kb - nl;
if j < 1, j = j + NB; end
dd = buf(:, j);
kb = kb + 1;
if kb > NB, kb = 1; end
trk = dd(7) > 0.5 && all(isfinite(dd(1:6)));
if trk
    pos = [dd(1); dd(2); dd(3); dd(6)];
end
if QD2_SIM.pose_onboard < 0.5
    pos = [x(1); x(2); x(3); x(9)];   % estimación ideal (solo para comparar)
    trk = true;
end
% velocidad: complementario acelerómetro + derivada de OptiTrack (LPF 2o orden
% wn = 50 rad/s, zeta = 1; Kp3 = 4), como HORIZON FRAME CONVERSION AND ESTIMATION
dpos = (pos(1:3) - pprev)/dt;
pprev = pos(1:3);
a = 50*dt;
vf1 = vf1 + a*(dpos - vf1);
vf2 = vf2 + a*(vf1 - vf2);
acc = ([x(4); x(5); x(6)] - vprev)/dt;
vprev = [x(4); x(5); x(6)];
vest = vest + dt*(acc + 4*(vf2 - vest));
if QD2_SIM.pose_onboard < 0.5
    vest = [x(4); x(5); x(6)];
end
x_est = [pos(1); pos(2); pos(3); vest(1); vest(2); vest(3); x(7); x(8); pos(4)];
% ---- errores del stack original (STATE MACHINE SIGNALS) ----------------
if ~trk && t > 1
    t_trk = t_trk + dt;
else
    t_trk = 0;
end
err_trk = t_trk >= 0.2;
err_com = t > 3 && t_com >= 0.5;
if (err_trk || err_com) && ob.fsm <= 6
    ob.fsm = 7;                % Error -> EMERGENCY STOP (rampa)
    T7 = u_prev(1);
end
if t_com >= 1.0 && tr(1) > 0.5 && ob.fsm ~= 9
    ob.fsm = 9;                % FLIGHT SAFETY: enlace perdido 1 s y armado -> corta motores
end
% ---- falla a bordo programada (QD2_SIM.falla_fsm [dron t]) o al estar apilados
% (QD2_SIM.falla_apilado: 1 = falla el de ARRIBA, 2 = el de ABAJO, tras 1 s con
% dh < 0.15 m y dz > 0.5 m): Error -> estado 7 como el stack original
falla = false;
fa = QD2_SIM.falla_fsm;
for k = 1:size(fa, 1)
    if fa(k,1) == ID && fa(k,2) >= 0 && t >= fa(k,2)
        falla = true;
    end
end
if QD2_SIM.falla_apilado > 0.5 && all(isfinite(mx(1:3)))
    dz = x(3) - mx(3);
    apil = sqrt((x(1) - mx(1))^2 + (x(2) - mx(2))^2) < 0.15 && abs(dz) > 0.5 && min(x(3), mx(3)) > 0.2;
    yo_arriba = dz > 0;
    if apil && ((QD2_SIM.falla_apilado < 1.5 && yo_arriba) || (QD2_SIM.falla_apilado > 1.5 && ~yo_arriba))
        t_ap = t_ap + dt;
    else
        t_ap = 0;
    end
    if t_ap >= 1.0
        falla = true;
    end
end
if falla && ~fh && ob.fsm >= 1 && ob.fsm <= 6
    fh = true;
    ob.fsm = 7;
    T7 = u_prev(1);
end
if tr(3) > 0.5
    ob.fsm = 9;                % E-stop: corte de motores (estado 8 -> 9 del original)
end
modo = 1;
if version > 1.5 && mx(7) > 0.5
    modo = 2;
end
otro = [mx(1); mx(2); mx(3); mx(4); mx(5); mx(6)];
ref = [ds(1) ds(2) ds(3) ds(4)];
if ob.fsm == 7
    % actitud nivelada, sin control de posición, empuje baja a 1.75 N/s
    T7 = max(T7 - 1.75*dt, 0);
    u = [T7; 0; 0; 0];
    if T7 <= 7.38
        ob.fsm = 9;
        u = zeros(4, 1);
    end
else
    [u, ob] = qd2_onboard_step(ob, tr(1), tr(2), ref, x_est, otro, QD2P, dt, modo);
end
u_prev = u;
bat = bat - dt*3.2e-4*u(1);   % descarga simple: ~0.005 V/s en hover
est = 3;
if ob.fsm >= 4 && ob.fsm <= 6
    if modo > 1.5
        est = ob.status;
    else
        est = 4;
    end
end
st = [ob.fsm; bat; est; u(1); double(err_com)];

== matlab function QD2_Sim_Dual/QDRONE 2 #2 (SIM)/ON-BOARD STACK (FSM + PIV or MPC) ==
  data: trig input; u output size=[4 1]; des input; mpcx input; x input; version input; dpose input; t input; st output size=[5 1]; QD2P parameter; QD2_SIM parameter
function [u, st] = fcn(trig, des, mpcx, x, version, dpose, t, QD2P, QD2_SIM)
%#codegen
% STACK A BORDO SIMULADO del QDrone 2 #2 (500 Hz): FSM + PIV original o MPC
% (qd2_onboard_step), con la estimación y los errores del stack real.
% trig = [arm takeoff estop 0], des = pose deseada [x y z yaw],
% mpcx = [otro dron x y z vx vy vz, mpc_mode, 0] (índices 17-24 del paquete MPC),
% x = estado verdadero de la planta (solo para la IMU: roll, pitch, aceleración),
% dpose = OptiTrack [x y z roll pitch yaw isTracking] (100 Hz, NaN sin rastreo).
ID = 2;
NB = 64;
persistent ob bat buf kb pos vf1 vf2 vest vprev pprev t_trk t_com paq T7 u_prev fh t_ap
dt = 0.002;
if isempty(ob)
    ob = qd2_onboard_init(QD2P);
    bat = 16.4;
    buf = zeros(7, NB);
    for j = 1:NB
        buf(:, j) = [x(1); x(2); x(3); x(7); x(8); x(9); 1];
    end
    kb = 1;
    pos = [x(1); x(2); x(3); x(9)];
    pprev = pos(1:3);
    vf1 = zeros(3, 1); vf2 = zeros(3, 1); vest = zeros(3, 1);
    vprev = [x(4); x(5); x(6)];
    t_trk = 0; t_com = 0; T7 = 0;
    paq = [trig(:); des(:); mpcx(:); dpose(:)];
    u_prev = zeros(4, 1);
    fh = false; t_ap = 0;
end
% ---- enlace PC -> dron: pérdidas programadas QD2_SIM.comm_off [dron t1 t2] ----
sin_enlace = false;
co = QD2_SIM.comm_off;
for k = 1:size(co, 1)
    if co(k,1) == ID && t >= co(k,2) && t < co(k,3)
        sin_enlace = true;
    end
end
if ~sin_enlace
    paq = [trig(:); des(:); mpcx(:); dpose(:)];   % "most recent": sin enlace queda el último
    t_com = 0;
else
    t_com = t_com + dt;
end
tr = paq(1:4); ds = paq(5:8); mx = paq(9:16); dp = paq(17:23);
% ---- estimación a bordo ------------------------------------------------
% pose OptiTrack con latencia (buffer circular a 500 Hz)
buf(:, kb) = dp;
nl = min(max(round(QD2_SIM.lat_pose/dt), 0), NB - 1);
j = kb - nl;
if j < 1, j = j + NB; end
dd = buf(:, j);
kb = kb + 1;
if kb > NB, kb = 1; end
trk = dd(7) > 0.5 && all(isfinite(dd(1:6)));
if trk
    pos = [dd(1); dd(2); dd(3); dd(6)];
end
if QD2_SIM.pose_onboard < 0.5
    pos = [x(1); x(2); x(3); x(9)];   % estimación ideal (solo para comparar)
    trk = true;
end
% velocidad: complementario acelerómetro + derivada de OptiTrack (LPF 2o orden
% wn = 50 rad/s, zeta = 1; Kp3 = 4), como HORIZON FRAME CONVERSION AND ESTIMATION
dpos = (pos(1:3) - pprev)/dt;
pprev = pos(1:3);
a = 50*dt;
vf1 = vf1 + a*(dpos - vf1);
vf2 = vf2 + a*(vf1 - vf2);
acc = ([x(4); x(5); x(6)] - vprev)/dt;
vprev = [x(4); x(5); x(6)];
vest = vest + dt*(acc + 4*(vf2 - vest));
if QD2_SIM.pose_onboard < 0.5
    vest = [x(4); x(5); x(6)];
end
x_est = [pos(1); pos(2); pos(3); vest(1); vest(2); vest(3); x(7); x(8); pos(4)];
% ---- errores del stack original (STATE MACHINE SIGNALS) ----------------
if ~trk && t > 1
    t_trk = t_trk + dt;
else
    t_trk = 0;
end
err_trk = t_trk >= 0.2;
err_com = t > 3 && t_com >= 0.5;
if (err_trk || err_com) && ob.fsm <= 6
    ob.fsm = 7;                % Error -> EMERGENCY STOP (rampa)
    T7 = u_prev(1);
end
if t_com >= 1.0 && tr(1) > 0.5 && ob.fsm ~= 9
    ob.fsm = 9;                % FLIGHT SAFETY: enlace perdido 1 s y armado -> corta motores
end
% ---- falla a bordo programada (QD2_SIM.falla_fsm [dron t]) o al estar apilados
% (QD2_SIM.falla_apilado: 1 = falla el de ARRIBA, 2 = el de ABAJO, tras 1 s con
% dh < 0.15 m y dz > 0.5 m): Error -> estado 7 como el stack original
falla = false;
fa = QD2_SIM.falla_fsm;
for k = 1:size(fa, 1)
    if fa(k,1) == ID && fa(k,2) >= 0 && t >= fa(k,2)
        falla = true;
    end
end
if QD2_SIM.falla_apilado > 0.5 && all(isfinite(mx(1:3)))
    dz = x(3) - mx(3);
    apil = sqrt((x(1) - mx(1))^2 + (x(2) - mx(2))^2) < 0.15 && abs(dz) > 0.5 && min(x(3), mx(3)) > 0.2;
    yo_arriba = dz > 0;
    if apil && ((QD2_SIM.falla_apilado < 1.5 && yo_arriba) || (QD2_SIM.falla_apilado > 1.5 && ~yo_arriba))
        t_ap = t_ap + dt;
    else
        t_ap = 0;
    end
    if t_ap >= 1.0
        falla = true;
    end
end
if falla && ~fh && ob.fsm >= 1 && ob.fsm <= 6
    fh = true;
    ob.fsm = 7;
    T7 = u_prev(1);
end
if tr(3) > 0.5
    ob.fsm = 9;                % E-stop: corte de motores (estado 8 -> 9 del original)
end
modo = 1;
if version > 1.5 && mx(7) > 0.5
    modo = 2;
end
otro = [mx(1); mx(2); mx(3); mx(4); mx(5); mx(6)];
ref = [ds(1) ds(2) ds(3) ds(4)];
if ob.fsm == 7
    % actitud nivelada, sin control de posición, empuje baja a 1.75 N/s
    T7 = max(T7 - 1.75*dt, 0);
    u = [T7; 0; 0; 0];
    if T7 <= 7.38
        ob.fsm = 9;
        u = zeros(4, 1);
    end
else
    [u, ob] = qd2_onboard_step(ob, tr(1), tr(2), ref, x_est, otro, QD2P, dt, modo);
end
u_prev = u;
bat = bat - dt*3.2e-4*u(1);   % descarga simple: ~0.005 V/s en hover
est = 3;
if ob.fsm >= 4 && ob.fsm <= 6
    if modo > 1.5
        est = ob.status;
    else
        est = 4;
    end
end
st = [ob.fsm; bat; est; u(1); double(err_com)];

== matlab function QD2_Sim_Dual/QDRONE 2 #2 (SIM)/PLANT (qd2_quad_plant) ==
  data: u input; x output size=[10 1]; F input; home input; QD2P parameter
function x = fcn(u, F, home, QD2P)
%#codegen
% PLANTA: qd2_quad_plant (traslación 3D, actitud y empuje de 1er orden, suelo).
persistent xs
if isempty(xs)
    xs = zeros(10, 1);
    xs(1) = home(1);
    xs(2) = home(2);
end
xs = qd2_quad_plant(xs, u, F, 0.002, QD2P.planta);
x = xs;

== matlab function QD2_Sim_Dual/DOWNWASH COUPLING/qd2_downwash (both ways) ==
  data: x1 input; F1 output size=[3 1]; x2 input; n input; F2 output size=[3 1]; QD2P parameter; QD2_SIM parameter
function [F1, F2] = fcn(x1, x2, n, QD2P, QD2_SIM)
%#codegen
% Downwash del dron de arriba sobre el de abajo (qd2_downwash) + turbulencia.
% QD2_SIM.dw_factor = downwash "real" / modelo del feedforward del MPC.
p1 = [x1(1) x1(2) x1(3)];
p2 = [x2(1) x2(2) x2(3)];
[Fa, sa] = qd2_downwash(p1, p2, QD2P.dw);
[Fb, sb] = qd2_downwash(p2, p1, QD2P.dw);
k = QD2_SIM.dw_factor;
F1 = k*(Fa + sa.*[n(1); n(2); n(3)]);
F2 = k*(Fb + sb.*[n(4); n(5); n(6)]);

== matlab function QD2_Sim_Dual/OPTITRACK (SIM, 100 Hz)/Measurement Conditioning (RSF) ==
  data: x1 input; d1 output size=[7 1]; x2 input; n input; t input; d2 output size=[7 1]; QD2_SIM parameter
function [d1, d2] = fcn(x1, x2, n, t, QD2_SIM)
%#codegen
% OptiTrack simulado: Corrected Pose Data [x y z roll pitch yaw isTracking]
% (mismo formato que Measurement Conditioning del MissionCtrl).
rp = QD2_SIM.ruido_pos; ry = QD2_SIM.ruido_yaw;
d1 = [x1(1) + rp*n(1); x1(2) + rp*n(2); x1(3) + rp*n(3); x1(7); x1(8); x1(9) + ry*n(4); 1];
d2 = [x2(1) + rp*n(5); x2(2) + rp*n(6); x2(3) + rp*n(7); x2(7); x2(8); x2(9) + ry*n(8); 1];
% pérdidas de rastreo programadas: filas [dron t1 t2]
tk = QD2_SIM.trk_off;
for i = 1:size(tk, 1)
    if t >= tk(i,2) && t < tk(i,3)
        if tk(i,1) == 1
            d1 = [nan(6,1); 0];
        elseif tk(i,1) == 2
            d2 = [nan(6,1); 0];
        end
    end
end

== matlab function QD2_Sim_Dual/SETPOINT SELECT (PID: GUARD, MPC: DIRECT) ==
  data: version input; sp1 output size=[4 1]; sp1_m input; sp2_m input; sp1_g input; sp2_g input; guard_g input; sp2 output size=[4 1]; guard output size=1
function [sp1, sp2, guard] = fcn(version, sp1_m, sp2_m, sp1_g, sp2_g, guard_g)
%#codegen
% PID: consignas del SEPARATION GUARD. MPC: consignas del supervisor (apilado
% permitido, el MPC a bordo compensa el downwash).
if version < 1.5
    sp1 = sp1_g; sp2 = sp2_g; guard = guard_g;
else
    sp1 = sp1_m; sp2 = sp2_m; guard = 0;
end
